simulink model "ESC_Motor"  (R2025b)
settings: Solver=FixedStepAuto  StartTime=0.0  StopTime=10.0  FixedStep=0.05  RelTol=1e-3
settings Model: Creator=FOFIEVIGOLBRYAN  LastModifiedBy=FOFIEVIGOLBRYAN

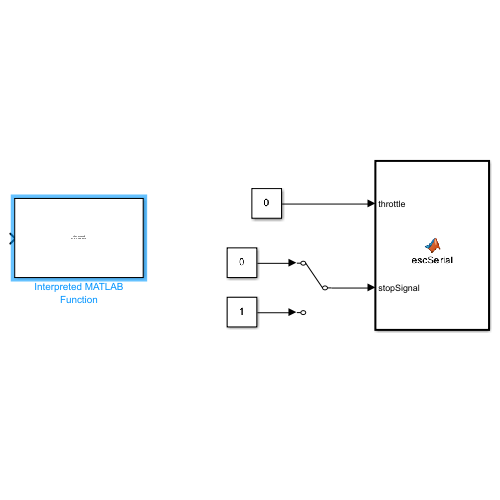
[thumbnail: Simulink's stored preview of the top-level diagram]
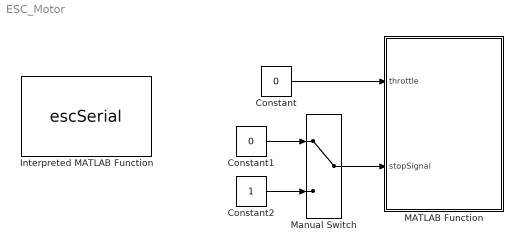
== system ESC_Motor ==
  Constant : Constant  Value=0
  Constant1 : Constant  Value=0
  Constant2 : Constant
  Interpreted MATLAB Function : MATLABFcn  MATLABFcn=escSerial  OutputDimensions=0
  MATLAB Function : MATLAB Function  TreatAsAtomicUnit=on
  Manual Switch : ManualSwitch
  wires:
  Constant/1 -> MATLAB Function/1(throttle)
  Manual Switch/1 -> MATLAB Function/2(stopSignal)
  Constant1/1 -> Manual Switch/1
  Constant2/1 -> Manual Switch/2

== matlab function ESC_Motor/MATLAB Function ==
  data: throttle input; stopSignal input
function escSerial(throttle, stopSignal)
% escSerial: envoie throttle (T,...) et stop (X) à l'ESP32 sur le même serialport

PORT = "COM8";
BAUD = 115200;

persistent sp lastSent wasStopped tLast
if isempty(sp)
    sp = serialport(PORT, BAUD);
    configureTerminator(sp, "LF");
    flush(sp);
    lastSent   = single(-1);
    wasStopped = false;
    tLast      = tic;
end

% ---- STOP prioritaire ----
if stopSignal ~= 0
    if ~wasStopped
        write(sp, "X\n", "string");
        wasStopped = true;
    end
    return; % si stop actif, on n'envoie pas de throttle
else
    wasStopped = false;
end

% ---- Throttle ----
% saturation 0..1
if throttle < 0
    throttle = 0;
elseif throttle > 1
    throttle = 1;
end
throttle = single(throttle);

% limiter fréquence d’envoi (20 Hz)
SEND_PERIOD = 0.05;
if toc(tLast) < SEND_PERIOD
    return;
end
tLast = tic;

% n’envoyer que si variation significative
if abs(throttle - lastSent) > 0.002
    cmd = sprintf("T,%.3f\n", throttle);
    write(sp, cmd, "string");
    lastSent = throttle;
end
end
